simulink model "tutorial32_pendulum"  (R2025a)
settings: Solver=VariableStepAuto  StartTime=0.0  StopTime=10.0  RelTol=1e-3
libraries: simulink x1
settings Model: Creator=xing2  LastModifiedBy=xing2

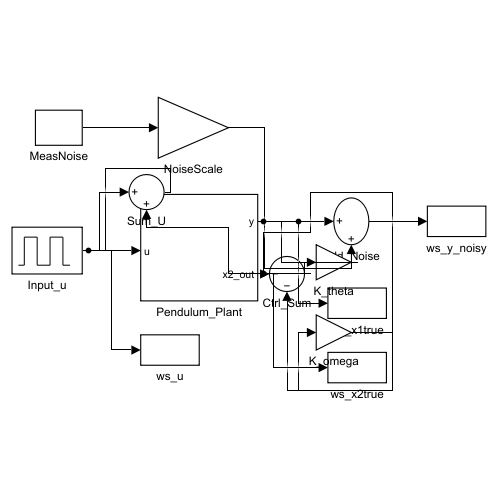
[thumbnail: Simulink's stored preview of the top-level diagram]
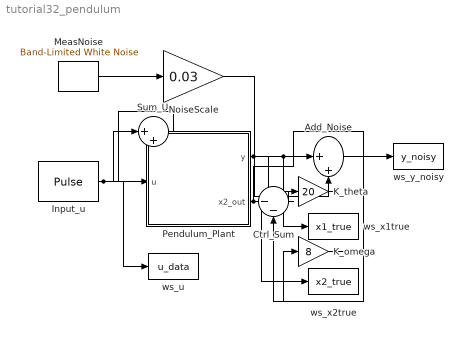
== system tutorial32_pendulum ==
  Add_Noise : Sum  Inputs=|++
  Ctrl_Sum : Sum  Inputs=|--
  Input_u : DiscretePulseGenerator  PulseType=Time based  Amplitude=0.3  Period=4  PulseWidth=25  PhaseDelay=0.5
  K_omega : Gain  Gain=8
  K_theta : Gain  Gain=20
  MeasNoise : simulink/Sources/Band-Limited White Noise  Cov=[0.1]  Ts=0.1  seed=[23341]
  NoiseScale : Gain  Gain=0.03
  Pendulum_Plant : Subsystem
  Sum_U : Sum  Inputs=|++
  ws_u : ToWorkspace  VariableName=u_data  SaveFormat=Timeseries  SampleTime=-1
  ws_x1true : ToWorkspace  VariableName=x1_true  SaveFormat=Timeseries  SampleTime=-1
  ws_x2true : ToWorkspace  VariableName=x2_true  SaveFormat=Timeseries  SampleTime=-1
  ws_y_noisy : ToWorkspace  VariableName=y_noisy  SaveFormat=Timeseries  SampleTime=-1
  wires:
  NoiseScale/1 -> Add_Noise/2
  Input_u/1 -> ws_u/1, Sum_U/1
  MeasNoise/1 -> NoiseScale/1
  Pendulum_Plant/2(x2_out) -> ws_x2true/1, K_omega/1
  Pendulum_Plant/1(y) -> Add_Noise/1, ws_x1true/1, K_theta/1
  Add_Noise/1 -> ws_y_noisy/1
  K_theta/1 -> Ctrl_Sum/1
  K_omega/1 -> Ctrl_Sum/2
  Ctrl_Sum/1 -> Sum_U/2
  Sum_U/1 -> Pendulum_Plant/1(u)

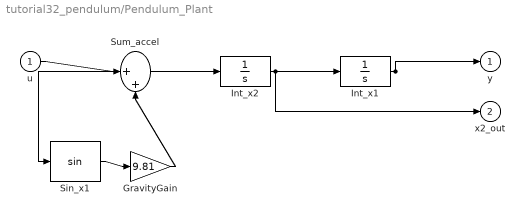
== system tutorial32_pendulum/Pendulum_Plant ==
  u : Inport
  GravityGain : Gain  Gain=9.81
  Int_x1 : Integrator  InitialCondition=0.5
  Int_x2 : Integrator
  Sin_x1 : Trigonometry
  Sum_accel : Sum  Inputs=|++
  y : Outport
  x2_out : Outport  Port=2
  wires:
  u/1 -> Sum_accel/1
  Sum_accel/1 -> Int_x2/1
  Int_x2/1 -> Int_x1/1, x2_out/1
  Int_x1/1 -> Sin_x1/1, y/1
  Sin_x1/1 -> GravityGain/1
  GravityGain/1 -> Sum_accel/2
